simulink model "Modello_Tesi_Capitolo5_ZOH"  (R2026b)
settings: Solver=ode15s  RelTol=1e-6  AbsTol=1e-8
values from neighbouring files (symbols this model uses):
  A = [Z, I_mat ... (first row only)    [Modello_Ago_Flessibile.m]    (also in test_morbido.m = [zeros(N, N), eye(N); test_rigido.m = [zeros(N, N), eye(N))
  A_kalman = sys.A - L_k * sys.C    [Modello_Ago_Flessibile.m]
  B_kalman = [Bu_base, L_k]    [Modello_Ago_Flessibile.m]
  Bu_base = sys.B(:, 1)    [Modello_Ago_Flessibile.m]
  C = zeros(1, 2*N)    [Modello_Ago_Flessibile.m]
  C_kalman = eye(n_stati)    [Modello_Ago_Flessibile.m]
  D_kalman = zeros(n_stati, 2)    [Modello_Ago_Flessibile.m]
  K_i = K_aug(end)    [Modello_Ago_Flessibile.m]    (also in tuning_LQR.m = K_aug(41))
  K_x = K_aug(1:n_stati)    [Modello_Ago_Flessibile.m]    (also in tuning_LQR.m = K_aug(1:40))
  x0_stimato = zeros(n_stati, 1)    [Modello_Ago_Flessibile.m]
libraries: simulink x1
settings Model: Creator=NICCOLO'  LastModifiedBy=NICCOLO'

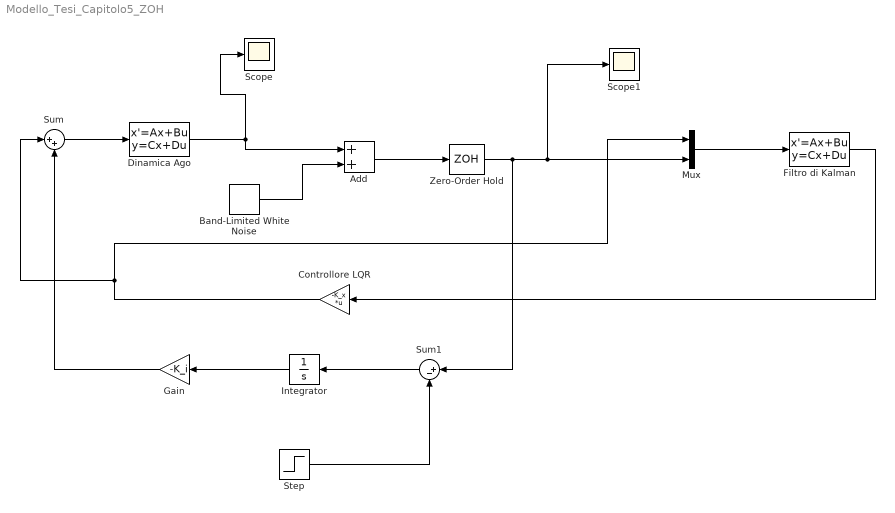
== system Modello_Tesi_Capitolo5_ZOH ==
  Add : Sum
  Band-Limited White Noise : simulink/Sources/Band-Limited White Noise  Cov=1e-9  Ts=0.033  seed=[23341]
  Controllore LQR : Gain  Gain=-K_x  Multiplication=Matrix(K*u)
  Dinamica Ago : StateSpace  A=A  B=Bu_base  C=C  D=0  InitialCondition=0  AllowTunableDMatrix=on
  Filtro di Kalman : StateSpace  A=A_kalman  B=B_kalman  C=C_kalman  D=D_kalman  InitialCondition=x0_stimato  AllowTunableDMatrix=on
  Gain : Gain  Gain=-K_i
  Integrator : Integrator
  Mux : Mux  Inputs=2
  Scope : Scope
      settings: ActiveDisplayYMinimum=-0.00067958701633737692  ActiveDisplayYMaximum=0.0057807296954321069
  Scope1 : Scope
      settings: ActiveDisplayYMinimum=-0.023898738959521028  ActiveDisplayYMaximum=0.060391604549976149
  Step : Step  Time=0.1  FinalValue=0.005  SampleTime=0
  Sum : Sum  Inputs=|++
  Sum1 : Sum  Inputs=|+-
  Zero-Order Hold : ZeroOrderHold  SampleTime=0.033
  wires:
  Dinamica Ago/1 -> Add/1, Scope/1
  Controllore LQR/1 -> Mux/1, Sum/1
  Mux/1 -> Filtro di Kalman/1
  Band-Limited White Noise/1 -> Add/2
  Add/1 -> Zero-Order Hold/1
  Zero-Order Hold/1 -> Sum1/1, Scope1/1, Mux/2
  Sum/1 -> Dinamica Ago/1
  Gain/1 -> Sum/2
  Step/1 -> Sum1/2
  Filtro di Kalman/1 -> Controllore LQR/1
  Integrator/1 -> Gain/1
  Sum1/1 -> Integrator/1
